simulink model "sds2204x_demo"  (R2022b)
settings: Solver=FixedStepAuto  StartTime=0.0  StopTime=inf  FixedStep=0.1  RelTol=1e-3
libraries: Links_TCP_Lib x3
settings Model: Creator=gao  LastModifiedBy=Administrator
settings SolverCC: AlgebraicLoopSolver=TrustRegion
settings OptimizationCC: BlockReduction=off
settings DebuggingCC: UnderspecifiedInitializationDetection=Classic  MergeDetectMultiDrivingBlocksExec=none  UnconnectedInputMsg=warning  UnconnectedOutputMsg=warning  UnconnectedLineMsg=warning  SFMachineParentedDataDiag=warning
settings HardwareCC: ProdBitPerLong=64  ProdHWDeviceType=Intel->x86-64 (Linux 64)
settings ModelReferenceCC: EnableRefExpFcnMdlSchedulingChecks=on  PropagateSignalLabelsOutOfModel=off
settings RTWCC: SystemTargetFile=links_rtlnx_grt.tlc  TemplateMakefile=links_rtlnx_grt.tmf
settings STFCustomTargetCC: TargetLangStandard=C99 (ISO)  CombineOutputUpdateFcns=on  SystemTargetFile=links_rtlnx_grt.tlc
settings GRTTargetCC: ParMdlRefBuildCompliant=off  CompOptLevelCompliant=off  ConcurrentExecutionCompliant=off  MatFileLogging=off  CPPClassGenCompliant=off  UseToolchainInfoCompliant=off  RTWCAPISignals=on  RTWCAPIParams=on  RTWCAPIRootIO=on

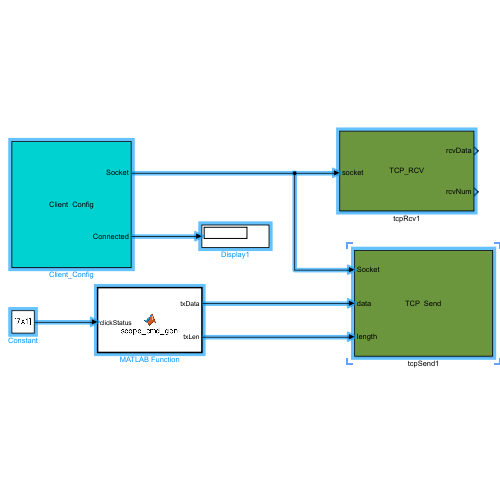
[thumbnail: Simulink's stored preview of the top-level diagram]
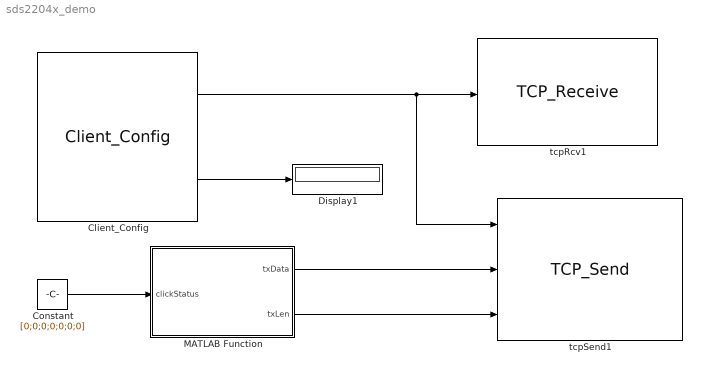
== system sds2204x_demo ==
  Client_Config : Links_TCP_Lib/Client_Config  serverIp=192.168.1.220  serverPort=5025  sampleTime=-1
      settings: SourceProductName=Links_LnxLib
  Constant : Constant  Value=[0;0;0;0;0;0;0]
  Display1 : Display
  MATLAB Function : MATLAB Function  TreatAsAtomicUnit=on
  tcpRcv1 : Links_TCP_Lib/TCP_Receive  width=32  sampletime=-1
      settings: SourceProductName=Links_LnxLib
  tcpSend1 : Links_TCP_Lib/TCP_Send  sampleTime=-1
      settings: SourceProductName=Links_LnxLib
  wires:
  Client_Config/2 -> Display1/1
  Client_Config/1 -> tcpSend1/1, tcpRcv1/1
  MATLAB Function/1(txData) -> tcpSend1/2
  Constant/1 -> MATLAB Function/1(clickStatus)
  MATLAB Function/2(txLen) -> tcpSend1/3

== matlab function sds2204x_demo/MATLAB Function ==
  data: txData output; clickStatus input; txLen output
function [txData, txLen] = scope_cmd_gen(clickStatus)
    % 示波器 SCPI 命令生成函数（无 values 版本）
    %
    % clickStatus: [1xN] double，UI 控件状态（0/1 或变化计数）
    %   1: NORMal/RUN     (开始运行,MODE NORMal)
    %   2: STOP    (停止/冻结)
    %   3: SINGLE  (单次触发)
    %   4: FTRIG  (强制触发)
    %   5: AUTO    (自动设置)
    %   6: 触发源=CH1 + 上升沿 (示例)
    %   7: 触发源=CH2 + 下降沿 (示例)
    %
    % txData: uint8 命令数组
    % txLen:  命令长度

    MAX_LEN = 64;
    LF = uint8(10);   % SCPI 结束符 \n
    
    txData = repmat(LF, 1, MAX_LEN);   % 全部填 0x0A
    txLen = int32(0);

    % 持久化变量（状态记忆）
    persistent prevClickStatus
    if isempty(prevClickStatus)
        prevClickStatus = zeros(7, 1);
    end

    
    cmd = uint8([]);  % 最终命令字节

    % --- 边缘检测：找第一个发生变化的按钮 ---
    diffStatus = clickStatus - prevClickStatus;
    changedIdx = 0;
    for k = 1:7
        if abs(diffStatus(k)) > 0
            changedIdx = k;
            break;
        end
    end

    % --- 根据变化的按钮组装 SCPI 命令 ---
    if changedIdx > 0
        switch changedIdx
            case 1 % NORMal
                  cmd = [uint8(':TRIGger:MODE NORMal'), LF];

            case 2 % STOP
                cmd = [uint8(':STOP'), LF];

            case 3 % SINGLE
                cmd = [uint8(':SINGLE'), LF];

            case 4 % 强制触发
                cmd = [uint8(':TRIGger:MODE FTRIG'), LF];

            case 5 % AUTO (自动设置)
                cmd = [uint8(':TRIGger:MODE AUTO'), LF];

            case 6 % 触发设置：CH1 上升沿
                cmd = [uint8(':TRIGger:EDGe:SOURce CHAN1'), LF, ...
                       uint8(':TRIGger:EDGe:SLOPe POSitive'), LF];

            case 7 % 触发设置：CH2 下降沿
                cmd = [uint8(':TRIGger:EDGe:SOURce CHAN2'), LF, ...
                       uint8(':TRIGger:EDGe:SLOPe NEGative'), LF];
        end
    end

    % --- 更新记忆 ---
    prevClickStatus = clickStatus;

    % --- 输出字节 ---
    txLen = int32(numel(cmd));
    if txLen > int32(MAX_LEN)
        txLen = int32(MAX_LEN);
    end
    if txLen > 0
        txData(1:txLen) = cmd(1:txLen);
    end

end
